simulink model "filtropasivoayudadios"  (R2023b)
settings: Solver=VariableStepAuto  StartTime=0.0  StopTime=10.0  RelTol=1e-3
libraries: fl_lib x5, nesl_utility x3, slctrl_linear x1
settings Model: Creator=Elias  LastModifiedBy=Elias

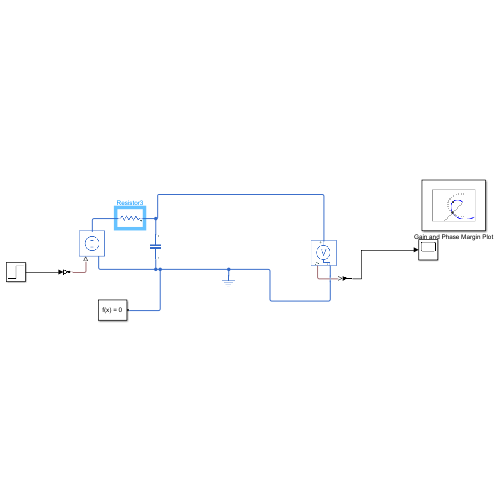
[thumbnail: Simulink's stored preview of the top-level diagram]
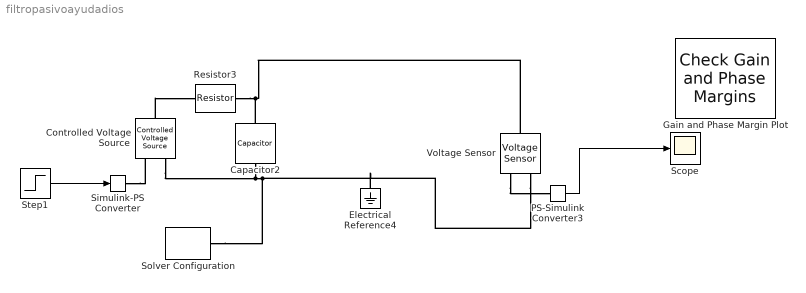
== system filtropasivoayudadios ==
  Capacitor2 : fl_lib/Electrical/Electrical Elements/Capacitor  c=2e-6 F  r=1e-9 Ohm  g=1e-9 1/Ohm  i_specify=off  i_priority=None  i=0 A  i_nominal_specify=off  i_nominal_unit=A  i_nominal_value=1  v_specify=off  v_priority=None  v=0 V  v_nominal_specify=off  v_nominal_unit=V  v_nominal_value=1  vc_specify=off  vc_priority=High  vc=0 V  vc_nominal_specify=off  vc_nominal_unit=V  vc_nominal_value=1
  Controlled Voltage Source : fl_lib/Electrical/Electrical Sources/Controlled Voltage Source
  Electrical Reference4 : fl_lib/Electrical/Electrical Elements/Electrical Reference
  Gain and Phase Margin Plot : slctrl_linear/Check Gain and Phase Margins  InstantiateOnLoad=on  SaveOperatingPoints=off  LinearizationIOs={'/Step1', 1, 'in', 'off', '';'/PS-Simulink Converter3', 1, 'out', 'on', ''}  LinearizeAt=SnapshotTimes  SnapshotTimes=[0]  TriggerType=rising  SampleTime=auto  RateConversionMethod=zoh  PreWarpFreq=10  UseExactDelayModel=off  UseFullBlockNameLabels=off  UseBusSignalLabels=off  enabled=on  stopWhenAssertionFail=off  export=off  ViewDlgPos=[1 49 1536 740.8]  LaunchViewOnOpen=off  OpenViewOnLoad=off  FrequencyUnits=rad/s  MagnitudeUnits=dB  PhaseUnits=deg  TimeUnits=seconds  EnableMargins=off  GainMargin=[]  PhaseMargin=[]  PlotType=bode  FeedbackSign=-1
      settings: LibrarySourceBlock=slctrlblks/Linear Analysis Plots/Gain and Phase Margin Plot  SaveToWorkspace=off  SaveName=sys
  PS-Simulink Converter3 : nesl_utility/PS-Simulink Converter  PhysicalDomain=network_engine_domain  SubClassName=ps_output  LeftPortType=input  RightPortType=output  PseudoPeriodic=off  Frequencies=[]  VectorFormat=inherit  Unit=inherit  AffineConversion=off
  Resistor3 : fl_lib/Electrical/Electrical Elements/Resistor  R=2 Ohm  i_specify=off  i_priority=None  i=0 A  i_nominal_specify=off  i_nominal_unit=A  i_nominal_value=1  v_specify=off  v_priority=None  v=0 V  v_nominal_specify=off  v_nominal_unit=V  v_nominal_value=1
  Scope : Scope
  Simulink-PS Converter : nesl_utility/Simulink-PS Converter  PhysicalDomain=network_engine_domain  SubClassName=ps_input  LeftPortType=input  RightPortType=output  PseudoPeriodic=off  Frequencies=[]  NoiseDistribution=none  NoiseParameters=[]  Unit=1  AffineConversion=on  FilteringAndDerivatives=filter  SimscapeFilterOrder=1  InputFilterTimeConstant=0.001  UdotUserProvided=0
  Solver Configuration : nesl_utility/Solver Configuration  PhysicalDomain=network_engine_domain  SubClassName=solver  LeftPortType=input  RightPortType=generic  Tones=[]  Harmonics=[]  SimulateNoise=off  Profile=off  UseLocalSampling=off  EnableSwitchedLinearOptims=on  FrequencyDomain=off  UseCCode=off  RelTol=0.001  AbsTol=0.001  MinStep=1e-09  ToWorkspace=off  RevertToSquareIcSolve=off  NumHomotopyIterations=100  PhasorMode=off  PhasorModeNumHarmonics=1  ConsistencySolver=NEWTON_XTOL_AFTER_FTOL  IndexReductionMethod=DerivativeReplacement  DoDC=off  ResidualTolerance=1e-09  ConsistencyTolSource=GLOBAL  ConsistencyAbsTol=0.001  ConsistencyRelTol=0.001  ConsistencyTolFactor=0.001  UseLocalSolver=off  LocalSolverChoice=NE_BACKWARD_EULER_ADVANCER  ResolveIndetEquations=on  FunctionEvalNumThread=1  LocalSolverSampleTime=0.001  DoFixedCost=off  MaxNonlinIter=3  MaxModeIter=2  ComputeImpulses=off  ImpulseIterations=2  LinearAlgebra=auto  LinearAlgebraNumThread=0  EquationFormulation=NE_TIME_EF  DelaysMemoryBudget=1024  AutomaticFiltering=on  FilteringTimeConstant=0.001  PartitionStorageMethod=AS_NEEDED  PartitionMemoryBudget=1024  PartitionMethod=ROBUST  MultibodyUseLocalSolver=off  MultibodyLocalSolverChoice=ODE1  MultibodyLocalSolverSampleTime=0.001
  Step1 : Step  SampleTime=0
  Voltage Sensor : fl_lib/Electrical/Electrical Sensors/Voltage Sensor
  wires:
  PS-Simulink Converter3/1 -> Scope/1
  Step1/1 -> Simulink-PS Converter/1
  connections:
  Controlled Voltage Source/RConn2 -- Capacitor2/RConn1 -- Voltage Sensor/RConn2 -- Electrical Reference4/LConn1 -- Solver Configuration/RConn1
  Voltage Sensor/RConn1 -- PS-Simulink Converter3/LConn1
  Simulink-PS Converter/RConn1 -- Controlled Voltage Source/RConn1
  Controlled Voltage Source/LConn1 -- Resistor3/RConn1
  Resistor3/LConn1 -- Voltage Sensor/LConn1 -- Capacitor2/LConn1
